simulink model "Ex4_Lista2_simul"  (R2025a)
settings: Solver=ode45  StartTime=0.0  StopTime=5  MaxStep=0.1  MinStep=0.1  RelTol=1e-3  EnableMultiTasking=on
values from neighbouring files (symbols this model uses):
  L = [0.5 0.5 0.2]    [Exc4_Lista2_code.m]
  ThetaA_0 = [-10 20 0]'    [Exc4_Lista2_code.m]
  W_0 = [1 2 3]    [Exc4_Lista2_code.m]
  XdotC0 = [-0.10 0 0]'    [Exc4_Lista2_code.m]
settings Model: Creator=aluno  LastModifiedBy=Gabriel Toledo
settings SolverCC: InitialStep=0.1  AlgebraicLoopSolver=TrustRegion
settings DataIOCC: LimitDataPoints=on  SaveFormat=Array  ReturnWorkspaceOutputs=off
settings OptimizationCC: LifeSpan=inf
settings DebuggingCC: SolverPrmCheckMsg=warning  UnconnectedInputMsg=warning  UnconnectedOutputMsg=warning  UnconnectedLineMsg=warning  SFUnexpectedBacktrackingDiag=warning  SFNoUnconditionalDefaultTransitionDiag=warning  SFExecutionAtInitializationDiag=none  ArithmeticOperatorsInVariantConditions=warning
settings HardwareCC: ProdBitPerPointer=32.0  ProdBitPerSizeT=32.0  ProdBitPerPtrDiffT=32.0  ProdLargestAtomicFloat=None  ProdIntDivRoundTo=Undefined  ProdEndianess=Unspecified  ProdWordSize=32.0  ProdHWDeviceType=32-bit Generic
settings ModelReferenceCC: PropagateSignalLabelsOutOfModel=off
settings SFSimCC: SimUseLocalCustomCode=off  CustomCodeUndefinedFunction=UseInterfaceOnly
settings RTWCC: RTWUseLocalCustomCode=off  GPUComputeCapability=3.5
settings CodeAppCC: StateflowObjectComments=on
settings GRTTargetCC: TargetLangStandard=C89/C90 (ANSI)
settings ConfigComp: CovMetricSettings=dw  CovSaveCumulativeToWorkspaceVar=on  CovSaveSingleToWorkspaceVar=on  CovExternalEMLEnable=off  CovSFcnEnable=off

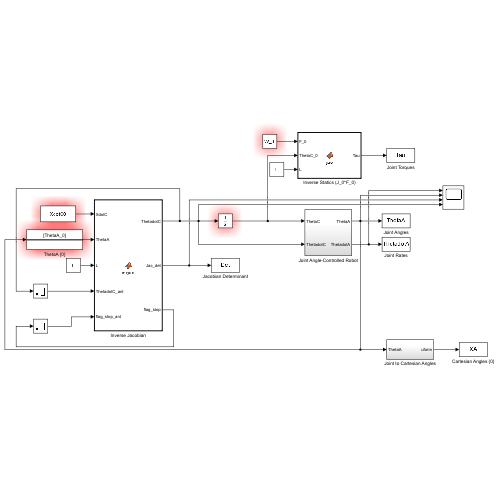
[thumbnail: Simulink's stored preview of the top-level diagram]
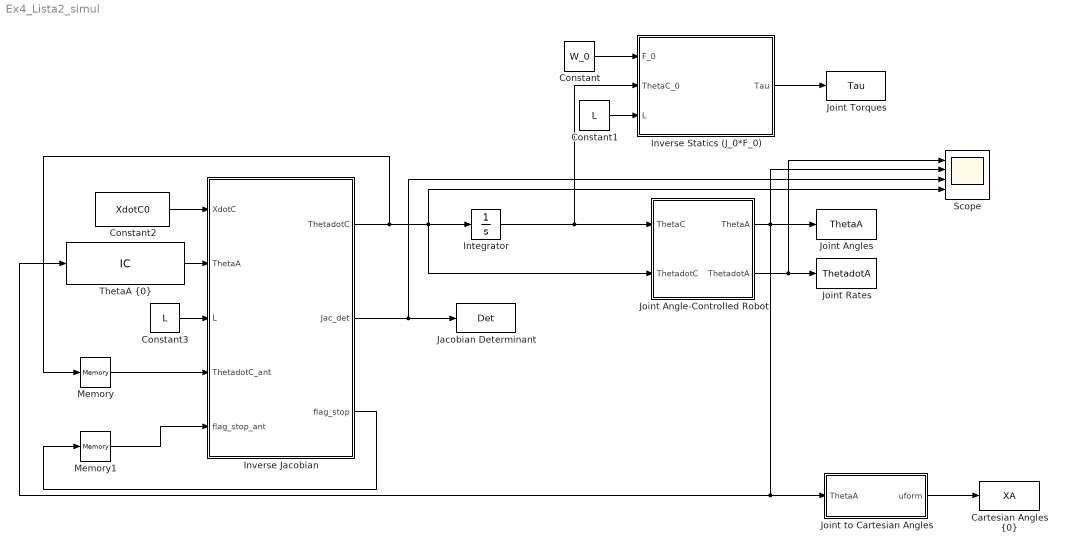
== system Ex4_Lista2_simul ==
  "Cartesian Angles {0}" : ToWorkspace  VariableName=XA  SaveFormat=Timeseries  SampleTime=-1
  Constant : Constant  Value=W_0
  Constant1 : Constant  Value=L
  Constant2 : Constant  Value=XdotC0
  Constant3 : Constant  Value=L
  Integrator : Integrator  InitialCondition=ThetaA_0
  Inverse Jacobian : MATLAB Function  TreatAsAtomicUnit=on
  Inverse Statics (J_0*F_0) : MATLAB Function  TreatAsAtomicUnit=on
  Jacobian Determinant : ToWorkspace  VariableName=Det  SaveFormat=Timeseries  SampleTime=-1
  Joint Angle-Controlled Robot : Subsystem
  Joint Angles : ToWorkspace  VariableName=ThetaA  SaveFormat=Timeseries  SampleTime=-1
  Joint Rates : ToWorkspace  VariableName=ThetadotA  SaveFormat=Timeseries  SampleTime=-1
  Joint Torques : ToWorkspace  VariableName=Tau  SaveFormat=Timeseries  SampleTime=-1
  Joint to Cartesian Angles : Subsystem
  Memory : Memory
  Memory1 : Memory
  Scope : Scope  NumInputPorts=4
      settings: ActiveDisplayYMinimum=-5  ActiveDisplayYMaximum=5  DataLoggingSaveFormat=Array
  "ThetaA {0}" : InitialCondition  Value=ThetaA_0
  wires:
  Constant3/1 -> Inverse Jacobian/3(L)
  Constant2/1 -> Inverse Jacobian/1(XdotC)
  Inverse Jacobian/1(ThetadotC) -> Memory/1, Joint Angle-Controlled Robot/2(ThetadotC), Scope/4, Integrator/1
  Inverse Jacobian/3(flag_stop) -> Memory1/1
  Inverse Jacobian/2(Jac_det) -> Scope/3, Jacobian Determinant/1
  "ThetaA {0}"/1 -> Inverse Jacobian/2(ThetaA)
  Integrator/1 -> Inverse Statics (J_0*F_0)/2(ThetaC_0), Joint Angle-Controlled Robot/1(ThetaC)
  Inverse Statics (J_0*F_0)/1(Tau) -> Joint Torques/1
  Joint Angle-Controlled Robot/2(ThetadotA) -> Scope/1, Joint Rates/1
  Joint Angle-Controlled Robot/1(ThetaA) -> Scope/2, Joint to Cartesian Angles/1(ThetaA), "ThetaA {0}"/1, Joint Angles/1
  Joint to Cartesian Angles/1(uform) -> "Cartesian Angles {0}"/1
  Constant/1 -> Inverse Statics (J_0*F_0)/1(F_0)
  Constant1/1 -> Inverse Statics (J_0*F_0)/3(L)
  Memory/1 -> Inverse Jacobian/4(ThetadotC_ant)
  Memory1/1 -> Inverse Jacobian/5(flag_stop_ant)

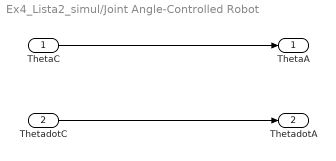
== system Ex4_Lista2_simul/Joint Angle-Controlled Robot ==
  ThetaC : Inport
  ThetadotC : Inport  Port=2
  ThetaA : Outport
  ThetadotA : Outport  Port=2
  wires:
  ThetaC/1 -> ThetaA/1
  ThetadotC/1 -> ThetadotA/1

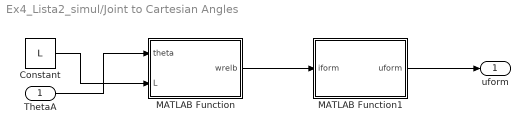
== system Ex4_Lista2_simul/Joint to Cartesian Angles ==
  ThetaA : Inport
  Constant : Constant  Value=L
  MATLAB Function : MATLAB Function  TreatAsAtomicUnit=on
  MATLAB Function1 : MATLAB Function  TreatAsAtomicUnit=on
  uform : Outport
  wires:
  ThetaA/1 -> MATLAB Function/1(theta)
  Constant/1 -> MATLAB Function/2(L)
  MATLAB Function/1(wrelb) -> MATLAB Function1/1(iform)
  MATLAB Function1/1(uform) -> uform/1

== matlab function Ex4_Lista2_simul/Inverse Statics (J_0*F_0) ==
  data: F_0 input; Tau output; ThetaC_0 input; L input
function Tau = jac(F_0, ThetaC_0, L)
%#codegen

J0 = [ -L(1)*sin(ThetaA(1)) - L(2)*sin(ThetaA(1)+ThetaA(2)), -L(2)*sin(ThetaA(1)+ThetaA(2)), 0;
       -L(1)*cos(ThetaA(1)) + L(2)*cos(ThetaA(1)+ThetaA(2)),  L(2)*cos(ThetaA(1)+ThetaA(2)), 0;
       1,                                                     1,                            1];

Tau = J0'*F_0;

end

== matlab function Ex4_Lista2_simul/Inverse Jacobian ==
  data: XdotC input; ThetadotC output; ThetaA input; L input; ThetadotC_ant input; flag_stop_ant input; Jac_det output; flag_stop output
function [ThetadotC, Jac_det, flag_stop]= invjac(XdotC, ThetaA, L, ThetadotC_ant, flag_stop_ant)
%#codegen

tolerance = 1e-6;

J0 = [ -L(1)*sind(ThetaA(1)) - L(2)*sind(ThetaA(1)+ThetaA(2)), -L(2)*sind(ThetaA(1)+ThetaA(2)), 0;
        L(1)*cosd(ThetaA(1)) + L(2)*cosd(ThetaA(1)+ThetaA(2)),  L(2)*cosd(ThetaA(1)+ThetaA(2)), 0;
       1,                                                       1,                             1];
   
Jac_det = det(J0);

flag_stop = flag_stop_ant;

if abs(Jac_det) < tolerance
    ThetadotC = ThetadotC_ant;
else
    inv_JO = J0^-1;
    ThetadotC = inv_JO*XdotC;
end

end

== matlab function Ex4_Lista2_simul/Joint to Cartesian Angles/MATLAB Function ==
  data: theta input; wrelb output; L input
%% Function
function wrelb = kin(theta, L)
%% Main Calculations

    Theta = theta(1) + theta(2) + theta(3);
    T = [cos(Theta)   -sin(Theta) 0 L(1)*cos(theta(1)) + L(2)*cos(theta(1) + theta(2));
         sin(Theta)    cos(Theta) 0 L(1)*sin(theta(1)) + L(2)*sin(theta(1) + theta(2));
         0              0           1 0;
         0              0           0 1];

%% Output Data

    wrelb = T;
    
end

== matlab function Ex4_Lista2_simul/Joint to Cartesian Angles/MATLAB Function1 ==
  data: iform input; uform output
%% Function
function uform = itou(iform)

%% Validity


%% Main Calculations

    theta = atan2(iform(2, 1),iform(1, 1));
    
    T = [iform(1, 4) iform(2, 4) theta];

%% Output Data

    uform = T;
    
end
